simulink model "ADCS_Simulink_FSW"  (R2025b)
settings: Solver=VariableStepAuto  StartTime=8000  StopTime=8700  FixedStep=0.001  RelTol=1e-3
PreLoadFcn:
  | addpath(genpath('../'))
  | adcsModelSetup();
values from neighbouring files (symbols this model uses):
  dT_Control = 1/10    (= 0.1)    [adcsModelSetup.m]
  fNoiseOn = 0    [adcsModelSetup.m]
undefined symbols (not defined in the file or in its folder): DiscIntNeverNeededParam, IAU, juliandate
libraries: vrlib x16, simulink_extras x7, sharedtransform x5, sharedutil x4, aerolibutil x4, sFunctionLibrary x4, simulink x3, matrix_library x2, aerolibtransform2 x2
(part 1 of 2)
settings Model: Creator=prani  LastModifiedBy=palla
settings DebuggingCC: ConsistencyChecking=warning  ArrayBoundsChecking=warning  CheckMatrixSingularityMsg=warning  ParameterUnderflowMsg=error  SFcnCompatibilityMsg=warning

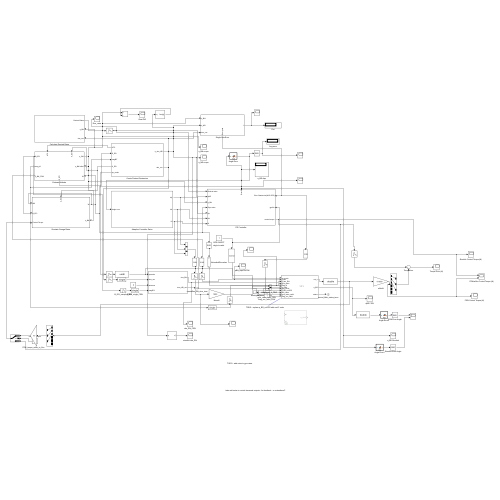
[thumbnail: Simulink's stored preview of the top-level diagram]
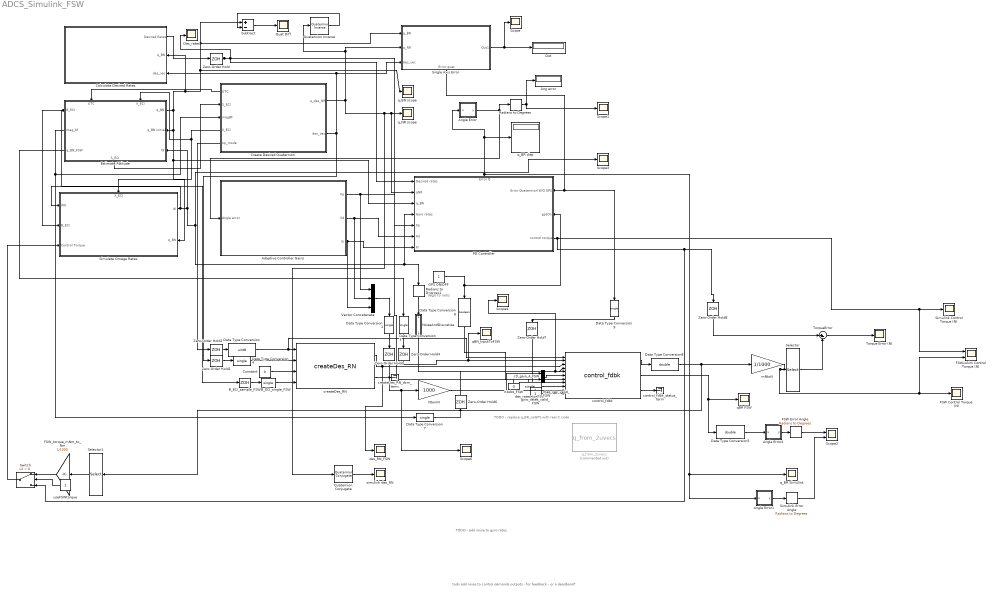
== system ADCS_Simulink_FSW ==
  note: todo add noise to control demands outputs - for feedback - or a deadband?
  note: TODO - add noise to gyro rates
  note: TODO - replace q_BR_noGPS with real C code
  note: deg/s to rad/s
  Adaptive Controller Gains : Subsystem
  Ang error : Display
  Angle Error : MATLAB Function  TreatAsAtomicUnit=on
  Angle Error1 : MATLAB Function  TreatAsAtomicUnit=on
  Angle Error2 : MATLAB Function  TreatAsAtomicUnit=on
  B_ECI_sample_FSW : ZeroOrderHold  SampleTime=dT_Control
  B_ECI_single_FSW : DataTypeConversion  OutDataTypeStr=single  SaturateOnIntegerOverflow=off  RndMeth=Floor
  Calculate Desired Rates : Subsystem
      settings: PortSchema="{\"entries\":[{\"content\":{\"sides\":[{\"content\":{},\"type\":\"ConnectorPlacement.EquallySpacedRectSide\",\"uuid\":\"787b8ffa-2bb6-4814-9cee-30d0a9949d62\"},{\"content\":{\"connectorIds\":[\"Out1\",\"In1\",\"In2\"],\"side\":\"RIGHT\"},\"type\":\"ConnectorPlacement.EquallySpacedRectSide\",\"uuid\":\"3e27d9b8-c1eb-4c63-90b1-636b0c297a4b\"},{\"content\":{\"side\":\"TOP\"},\"type\":\"ConnectorPlacement.EquallySpacedRectSide\",\"uuid\":\"66d7efb2-8eb7-483d-b673-bec0e962b7d7\"}]},\"type\":\"ConnectorPlacement.EquallySpacedConnector\",\"uuid\":\"bfb47682-ffbd-402c-af6d-784f4b216212\"}],\"packageUris\":[\"http://schema.mathworks.com/mf0/Connector/R2020b\"],\"version\":\"1.0\"}"
  Constant : Constant  Value=0  OutDataTypeStr=uint8
  Create Desired Quaternion : Subsystem
      settings: PortSchema="{\"entries\":[{\"content\":{\"sides\":[{\"content\":{\"connectorIds\":[\"Out3\",\"In1\",\"In2\",\"Out4\",\"Out5\"]},\"type\":\"ConnectorPlacement.EquallySpacedRectSide\",\"uuid\":\"a06b4b20-baa8-4cd2-8731-8e2324dbb8fc\"},{\"content\":{\"connectorIds\":[\"Out1\",\"Out2\"],\"side\":\"RIGHT\"},\"type\":\"ConnectorPlacement.EquallySpacedRectSide\",\"uuid\":\"e89e67ff-4894-42c1-b3ac-017f3fc977aa\"},{\"content\":{\"side\":\"TOP\"},\"type\":\"ConnectorPlacement.EquallySpacedRectSide\",\"uuid\":\"6ee5ea32-5253-456a-b6dd-ef60fd48a9e3\"}]},\"type\":\"ConnectorPlacement.EquallySpacedConnector\",\"uuid\":\"b732bf39-7b48-418d-8437-db30d99856db\"}],\"packageUris\":[\"http://schema.mathworks.com/mf0/Connector/R2020b\"],\"version\":\"1.0\"}"
  Data Type Conversion : DataTypeConversion  OutDataTypeStr=uint8  SaturateOnIntegerOverflow=off  RndMeth=Floor
  Data Type Conversion{1,3..4,7,9} (5 alike) : DataTypeConversion  OutDataTypeStr=single  SaturateOnIntegerOverflow=off  RndMeth=Floor
  Data Type Conversion5 : DataTypeConversion  OutDataTypeStr=double  SaturateOnIntegerOverflow=off  RndMeth=Floor
  Data Type Conversion6 : DataTypeConversion  OutDataTypeStr=boolean  SaturateOnIntegerOverflow=off  RndMeth=Floor
  Data Type Conversion8 : DataTypeConversion  OutDataTypeStr=double  SaturateOnIntegerOverflow=off  RndMeth=Floor
  Des_rates : Scope
      settings: ActiveDisplayYMinimum=-7.5812097384350083E-16  ActiveDisplayYMaximum=1.8036722603787631E-16  DataLoggingVariableName=ScopeData11
  Dot : Display
  Estimate Attitude : Subsystem
      settings: PortSchema="{\"entries\":[{\"content\":{\"sides\":[{\"content\":{\"connectorIds\":[\"Out3\",\"Out4\",\"Out5\"]},\"type\":\"ConnectorPlacement.EquallySpacedRectSide\",\"uuid\":\"9e22cb63-f739-4def-bc16-8f5ac96da1b2\"},{\"content\":{\"connectorIds\":[\"Out1\",\"In3\",\"In4\"],\"side\":\"RIGHT\"},\"type\":\"ConnectorPlacement.EquallySpacedRectSide\",\"uuid\":\"185e8ae2-f047-4dfe-b4b8-b24ace8a5036\"},{\"content\":{\"connectorIds\":[\"In1\",\"In2\"],\"side\":\"TOP\"},\"type\":\"ConnectorPlacement.EquallySpacedRectSide\",\"uuid\":\"aba5f04b-f2ef-4373-8d95-838bf2fc0f7e\"},{\"content\":{\"connectorIds\":[\"Out2\"],\"side\":\"BOTTOM\"},\"type\":\"ConnectorPlacement.EquallySpacedRectSide\",\"uuid\":\"34d3ae2b-3f47-4699-99b9-a603dee72b74\"}]},\"type\":\"ConnectorPlacement.EquallySpacedConnector\",\"uuid\":\"020a8ac0-54fe-466e-8166-8e2d9bca8ffa\"}],\"packageUris\":[\"http://schema.mathworks.com/mf0/Connector/R2020b\"],\"version\":\"1.0\"}"
  FSW Control Torque (N) : Scope
      settings: ActiveDisplayYMinimum=-0.1409447193145752  ActiveDisplayYMaximum=0.096963930130004886  DataLoggingVariableName=ScopeData30
  FSW Error Angle : simulink_extras/Transformations/Radians to Degrees
  FSW_torque_mNm_to_Nm : Gain  Gain=1/1000  OutDataTypeStr=double
  FSWvsSim Control Torque (N) : Scope  NumInputPorts=2
      settings: ActiveDisplayYMinimum=-0.021514837503433224  ActiveDisplayYMaximum=0.085270786523818975  DataLoggingVariableName=ScopeData45
  GPS ON/OFF : Constant
  Kbdot_FSW : Constant  Value=0  OutDataTypeStr=single  SampleTime=dT_Control
  NoiseAndDiscretise : Subsystem  mask{Mean=[0;0;0];, Variance=0.1*ones(3,1);, dT=dT_Control, fNoiseOn=1}
      mask prompts: fNoiseOn "Noise On (1/0)"
  NtomN : Gain  Gain=1000  OutDataTypeStr=single
  PD Controller : Subsystem
      settings: PortSchema="{\"entries\":[{\"content\":{\"sides\":[{\"content\":{\"connectorIds\":[\"In1\",\"In2\",\"In3\",\"In4\",\"In5\",\"In6\",\"In7\"]},\"type\":\"ConnectorPlacement.EquallySpacedRectSide\",\"uuid\":\"e7cfb03b-fdce-49bd-b114-b6383fec3453\"},{\"content\":{\"connectorIds\":[\"In8\",\"In9\",\"Out1\"],\"side\":\"RIGHT\"},\"type\":\"ConnectorPlacement.EquallySpacedRectSide\",\"uuid\":\"354243bd-d6fe-41fe-9aaf-62ec8dd6b288\"},{\"content\":{\"connectorIds\":[\"Out2\"],\"side\":\"TOP\"},\"type\":\"ConnectorPlacement.EquallySpacedRectSide\",\"uuid\":\"5bccfe41-e6a5-4734-99aa-97d0c6c76924\"}]},\"type\":\"ConnectorPlacement.EquallySpacedConnector\",\"uuid\":\"9d160725-4233-4f19-a31f-b456d9eba014\"}],\"packageUris\":[\"http://schema.mathworks.com/mf0/Connector/R2020b\"],\"version\":\"1.0\"}"
  Quat Diff : Scope
      settings: ActiveDisplayYMinimum=-2.4278695362681826  ActiveDisplayYMaximum=3.4846862195685198
  Quaternion Conjugate : aerolibutil/Quaternion Conjugate
  Quaternion Inverse : aerolibutil/Quaternion Inverse
  Radians to Degrees : simulink_extras/Transformations/Radians to Degrees
  Radians to Degrees1 : simulink_extras/Transformations/Radians to Degrees
  Scope{,1,3..4,6} (5 alike) : Scope
      Scope settings: ActiveDisplayYMinimum=-1.3627045234786557  ActiveDisplayYMaximum=1.3194577353207935  DataLoggingVariableName=ScopeData20
      Scope1 settings: ActiveDisplayYMinimum=-45.683444261397909  ActiveDisplayYMaximum=242.34455590666121
      Scope3 settings: ActiveDisplayYMinimum=-0.32288965159303823  ActiveDisplayYMaximum=0.19416046551698385  DataLoggingVariableName=ScopeData14
      Scope4 settings: ActiveDisplayYMinimum=-18.264092922210693  ActiveDisplayYMaximum=12.284894466400146  DataLoggingVariableName=ScopeData46
      Scope6 settings: ActiveDisplayYMinimum=-0.062499999999999986  ActiveDisplayYMaximum=0.5625  DataLoggingVariableName=ScopeData32
  Scope2 : Scope  NumInputPorts=2
      settings: ActiveDisplayYMinimum=-18.982567049476042  ActiveDisplayYMaximum=182.17965657034267  DataLoggingVariableName=ScopeData36
  Selector : Selector  InputPortWidth=6  IndexOptions=Index vector (dialog)  Indices=[1 2 3]  OutputSizes=1
  Selector1 : Selector  InputPortWidth=6  IndexOptions=Index vector (dialog)  Indices=[1 2 3]  OutputSizes=1
  Simulate Omega Rates : Subsystem
      settings: PortSchema="{\"entries\":[{\"content\":{\"sides\":[{\"content\":{\"connectorIds\":[\"In1\",\"In2\",\"In3\"]},\"type\":\"ConnectorPlacement.EquallySpacedRectSide\",\"uuid\":\"e90ec8a0-4b74-4e10-b2a7-e5fd2ae1e771\"},{\"content\":{\"connectorIds\":[\"Out1\",\"In5\"],\"side\":\"RIGHT\"},\"type\":\"ConnectorPlacement.EquallySpacedRectSide\",\"uuid\":\"99d2540c-d7ae-4cc6-9c8c-9f3376bc2204\"},{\"content\":{\"connectorIds\":[\"In4\"],\"side\":\"TOP\"},\"type\":\"ConnectorPlacement.EquallySpacedRectSide\",\"uuid\":\"1bb08a9c-3229-4768-9d5b-a9b542d9af4a\"},{\"content\":{\"side\":\"BOTTOM\"},\"type\":\"ConnectorPlacement.EquallySpacedRectSide\",\"uuid\":\"162a9998-95a8-4725-8cf6-c5c7f5c27aaf\"}]},\"type\":\"ConnectorPlacement.EquallySpacedConnector\",\"uuid\":\"560ef827-5a28-40b0-8e31-165022fcc335\"}],\"packageUris\":[\"http://schema.mathworks.com/mf0/Connector/R2020b\"],\"version\":\"1.0\"}"
  Simulink Control Torque (N) : Scope
      settings: ActiveDisplayYMinimum=-0.19285196494450457  ActiveDisplayYMaximum=0.22481895277845004  DataLoggingVariableName=ScopeData6
  Simulink Error Angle : simulink_extras/Transformations/Radians to Degrees
  Single Axis Error : Subsystem
      settings: PortSchema="{\"entries\":[{\"content\":{\"sides\":[{\"content\":{\"connectorIds\":[\"In1\",\"In2\",\"In3\"]},\"type\":\"ConnectorPlacement.EquallySpacedRectSide\",\"uuid\":\"b8267f91-c5e3-4d33-8203-7c1a132bc190\"},{\"content\":{\"connectorIds\":[\"Out1\"],\"side\":\"RIGHT\"},\"type\":\"ConnectorPlacement.EquallySpacedRectSide\",\"uuid\":\"66851e38-bd34-4725-8451-fc4e99cb0cf9\"},{\"content\":{\"side\":\"TOP\"},\"type\":\"ConnectorPlacement.EquallySpacedRectSide\",\"uuid\":\"dfe73cc2-180d-42b0-a8bc-469053aa0085\"},{\"content\":{\"connectorIds\":[\"Out2\"],\"side\":\"BOTTOM\"},\"type\":\"ConnectorPlacement.EquallySpacedRectSide\",\"uuid\":\"e4419c1d-78c1-4c02-89c9-5404581220d5\"}]},\"type\":\"ConnectorPlacement.EquallySpacedConnector\",\"uuid\":\"596ae20b-822c-4bb8-8293-fd61ff3bd564\"}],\"packageUris\":[\"http://schema.mathworks.com/mf0/Connector/R2020b\"],\"version\":\"1.0\"}"
  Subtract : Sum  Inputs=+-
  Switch : Switch  Criteria=u2 > Threshold  SaturateOnIntegerOverflow=off  InputSameDT=off
  Torque Error (N) : Scope
      settings: ActiveDisplayYMinimum=-0.015390724559551172  ActiveDisplayYMaximum=0.017866098622383832  DataLoggingVariableName=ScopeData31
  TorqueError : Sum  Inputs=|+-
  Vector Concatenate : Concatenate  NumInputs=3
  Zero-Order Hold : ZeroOrderHold
  Zero-Order Hold{1..4,6..8} (7 alike) : ZeroOrderHold  SampleTime=dT_Control
  control_fdbk : sFunctionLibrary/control_fdbk  SystemSampleTime=-1  VariantActivationTime=update diagram  EmptyChoice=off  PassThrough=off  PassThroughVariantControl=(default)  EmptyChoiceVariantControl=(default)  AllowFlexibleInterface=on  Latency=0  AutoFrameSizeCalculation=off
  control_fdbk_status_term : Terminator
  createDes_RN : sFunctionLibrary/createDes_RN  SystemSampleTime=-1  VariantActivationTime=update diagram  EmptyChoice=off  PassThrough=off  PassThroughVariantControl=(default)  EmptyChoiceVariantControl=(default)  AllowFlexibleInterface=on  Latency=0  AutoFrameSizeCalculation=off
  createDes_RN_dcm_term : Terminator
  ctl_gain_4_FSW : Concatenate
  des_RN_FSW : Scope
      settings: ActiveDisplayYMinimum=-1.2834040716711121  ActiveDisplayYMaximum=1.1693099245008391  DataLoggingVariableName=ScopeData33
  des_rates_to_FSW : DataTypeConversion  OutDataTypeStr=single  SaturateOnIntegerOverflow=off  RndMeth=Floor
  gyro_rates_valid_FSW : Constant  OutDataTypeStr=int32  SampleTime=dT_Control
  mNtoN : Gain  Gain=1/1000  OutDataTypeStr=double
  mag_vec_valid_FSW : Constant  OutDataTypeStr=int32  SampleTime=dT_Control
  qBN_InputToFSW : Scope
      settings: ActiveDisplayYMinimum=-1.1772833690047264  ActiveDisplayYMaximum=1.2419203743338585  DataLoggingVariableName=ScopeData41
  qBR FSW : Scope
      settings: ActiveDisplayYMinimum=-0.87164634466171265  ActiveDisplayYMaximum=1.2077648043632507  DataLoggingVariableName=ScopeData35
  q_BN scope : Scope
      settings: ActiveDisplayYMinimum=-1.3505009914765778  ActiveDisplayYMaximum=1.1663107803216415  DataLoggingVariableName=ScopeData4
  q_BR Simulink : Scope
      settings: ActiveDisplayYMinimum=-0.87279489122515741  ActiveDisplayYMaximum=1.2079931709273608  DataLoggingVariableName=ScopeData28
  q_BR disp : Display
  q_NR scope : Scope
      settings: ActiveDisplayYMinimum=-0.18271803790267854  ActiveDisplayYMaximum=0.94151609942253189  DataLoggingVariableName=ScopeData18
  q_from_2uvecs : sFunctionLibrary/q_from_2uvecs  Commented=on  SystemSampleTime=-1  VariantActivationTime=update diagram  EmptyChoice=off  PassThrough=off  PassThroughVariantControl=(default)  EmptyChoiceVariantControl=(default)  AllowFlexibleInterface=on  Latency=0  AutoFrameSizeCalculation=off
  simulink des_RN : Scope
      settings: ActiveDisplayYMinimum=-1.2267552075477972  ActiveDisplayYMaximum=1.2259656861469523  DataLoggingVariableName=ScopeData34
  useFSWtorque : Constant
  wires:
  Simulate Omega Rates/1(W) -> Scope3/1, PD Controller/4(Gyro rates), Radians to Degrees1/1, Estimate Attitude/4(W), Simulate Omega Rates/1(W0)
  Create Desired Quaternion/1(q_des_NR) -> Single Axis Error/2(q_NR), Quaternion Inverse/1, Quaternion Conjugate/1, q_NR scope/1, PD Controller/2(qNR)
  Single Axis Error/1(Out1) -> Scope/1, Dot/1
  Calculate Desired Rates/1(Desired Rates) -> Zero-Order Hold/1
  Adaptive Controller Gains/1(Kp) -> Vector Concatenate/1, PD Controller/5(Kp)
  Adaptive Controller Gains/2(Kd) -> Vector Concatenate/2, PD Controller/6(Kd)
  Adaptive Controller Gains/3(Ki) -> Vector Concatenate/3, PD Controller/7(Ki)
  Radians to Degrees/1 -> Scope1/1, Ang error/1
  Estimate Attitude/1(q_BN) -> PD Controller/3(q_BN), Simulate Omega Rates/5(q_BN), Estimate Attitude/3(q_BN initial), Calculate Desired Rates/1(q_BN), Subtract/1, Single Axis Error/1(q_BN), q_BN scope/1
  Quaternion Inverse/1 -> Subtract/2
  Subtract/1 -> Quat Diff/1
  Zero-Order Hold/1 -> Des_rates/1, PD Controller/1(Desired rates), des_rates_to_FSW/1
  Single Axis Error/2(Error quat) -> Data Type Conversion9/1, PD Controller/8(Error Quaternion(W/O GPS))
  Create Desired Quaternion/4(X_ECI) -> Estimate Attitude/2(X_ECI), Simulate Omega Rates/4(X_ECI)
  Create Desired Quaternion/3(UTC) -> Estimate Attitude/1(UTC)
  Estimate Attitude/2(S_ECI) -> Create Desired Quaternion/1(S_ECI)
  Create Desired Quaternion/2(des_vec) -> Single Axis Error/3(des_vec), Calculate Desired Rates/2(des_vec), Zero-Order Hold1/1
  Estimate Attitude/3(B_ECI) -> Simulate Omega Rates/2("B_ECI "), B_ECI_sample_FSW/1
  Create Desired Quaternion/5(op_mode) -> Zero-Order Hold2/1
  createDes_RN/1 -> des_RN_FSW/1, control_fdbk/3
  Vector Concatenate/1 -> Data Type Conversion1/1
  Angle Error/1(y) -> Radians to Degrees/1, Adaptive Controller Gains/1(Angle error)
  control_fdbk/1 -> Data Type Conversion8/1
  Data Type Conversion/1 -> createDes_RN/1, control_fdbk/1
  Data Type Conversion1/1 -> Zero-Order Hold3/1
  Data Type Conversion3/1 -> Zero-Order Hold4/1
  Zero-Order Hold1/1 -> Data Type Conversion4/1
  Zero-Order Hold2/1 -> Data Type Conversion/1
  Zero-Order Hold3/1 -> Scope6/1, NtomN/1
  Zero-Order Hold4/1 -> qBN_InputToFSW/1, control_fdbk/2
  Zero-Order Hold8/1 -> TorqueError/1
  TorqueError/1 -> Torque Error (N)/1
  Estimate Attitude/4(mag_bf) -> Create Desired Quaternion/2(magBF), Data Type Conversion7/1
  Data Type Conversion7/1 -> Zero-Order Hold6/1
  Data Type Conversion8/1 -> Selector1/1, mNtoN/1
  Quaternion Conjugate/1 -> simulink des_RN/1
  Data Type Conversion4/1 -> createDes_RN/2
  Constant/1 -> createDes_RN/3
  Zero-Order Hold6/1 -> control_fdbk/5
  control_fdbk/2 -> qBR FSW/1, Data Type Conversion5/1
  mNtoN/1 -> FSWvsSim Control Torque (N)/2, FSW Control Torque (N)/1, Selector/1
  Selector/1 -> TorqueError/2
  Angle Error2/1(y) -> FSW Error Angle/1
  Angle Error1/1(y) -> Simulink Error Angle/1
  Simulink Error Angle/1 -> Scope2/2
  FSW Error Angle/1 -> Scope2/1
  Data Type Conversion5/1 -> Angle Error2/1(u)
  NoiseAndDiscretise/1(Out1) -> Scope4/1, control_fdbk/4
  Radians to Degrees1/1 -> NoiseAndDiscretise/1(In1)
  Estimate Attitude/5(q_BN_FSW) -> Data Type Conversion3/1
  PD Controller/1(control torque) -> FSWvsSim Control Torque (N)/1, Simulink Control Torque (N)/1, Switch/3, Zero-Order Hold8/1
  GPS ON/OFF/1 -> Data Type Conversion6/1, PD Controller/9(gpsOn)
  Data Type Conversion6/1 -> control_fdbk/7
  PD Controller/2(Error Q) -> q_BR Simulink/1, Angle Error1/1(u), Angle Error/1(u), q_BR disp/1
  Zero-Order Hold7/1 -> control_fdbk/8
  Data Type Conversion9/1 -> Zero-Order Hold7/1
  Switch/1 -> Simulate Omega Rates/3(Control Torque)
  useFSWtorque/1 -> Switch/2
  des_rates_to_FSW/1 -> control_fdbk/9
  gyro_rates_valid_FSW/1 -> control_fdbk/10
  mag_vec_valid_FSW/1 -> control_fdbk/11
  control_fdbk/3 -> control_fdbk_status_term/1
  createDes_RN/2 -> createDes_RN_dcm_term/1
  NtomN/1 -> ctl_gain_4_FSW/1
  Kbdot_FSW/1 -> ctl_gain_4_FSW/2
  ctl_gain_4_FSW/1 -> control_fdbk/6
  B_ECI_sample_FSW/1 -> B_ECI_single_FSW/1
  B_ECI_single_FSW/1 -> createDes_RN/4
  Selector1/1 -> FSW_torque_mNm_to_Nm/1
  FSW_torque_mNm_to_Nm/1 -> Switch/1

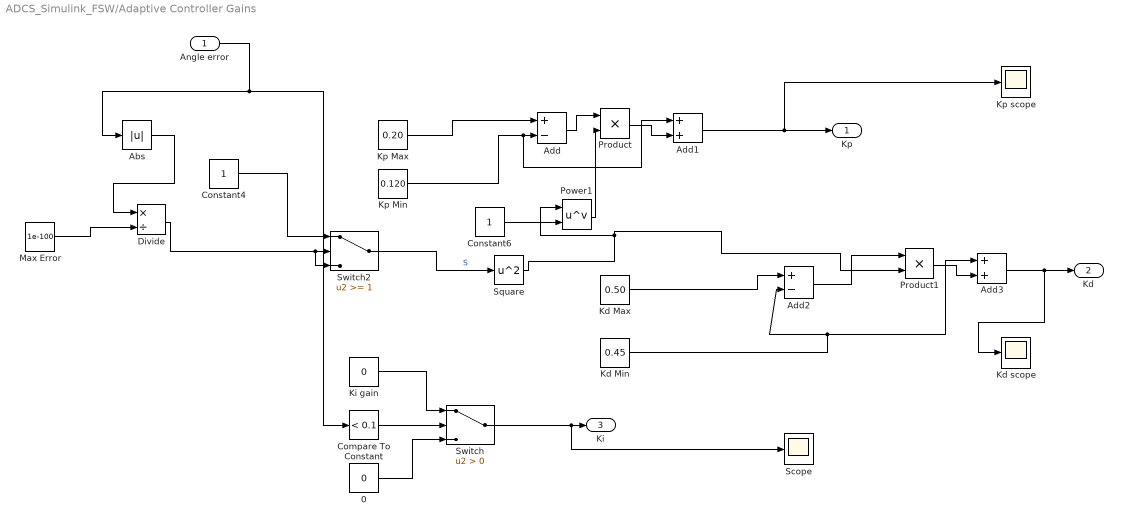
== system ADCS_Simulink_FSW/Adaptive Controller Gains ==
  Angle error : Inport
  0 : Constant  Value=0
  Abs : Abs  SaturateOnIntegerOverflow=off
  Add : Sum  Inputs=+-
  Add1 : Sum
  Add2 : Sum  Inputs=+-
  Add3 : Sum
  Compare To Constant : simulink/Logic and Bit Operations/Compare To Constant  relop=<  const=0.1  OutDataTypeStr=boolean
  Constant4 : Constant
  Constant6 : Constant
  Divide : Product  Inputs=*/
  Kd Max : Constant  Value=0.50
  Kd Min : Constant  Value=0.45
  Kd scope : Scope
      settings: ActiveDisplayYMinimum=0.4  ActiveDisplayYMaximum=0.6  DataLoggingVariableName=ScopeData3
  Ki gain : Constant  Value=0
  Kp Max : Constant  Value=0.20  VectorParams1D=off
  Kp Min : Constant  Value=0.120
  Kp scope : Scope
      settings: ActiveDisplayYMinimum=0.1  ActiveDisplayYMaximum=0.30000000000000004  DataLoggingVariableName=ScopeData5
  Max Error : Constant  Value=1e-100
  Power1 : Math  Operator=pow
  Product : Product
  Product1 : Product
  Scope : Scope
      settings: DataLoggingVariableName=ScopeData2
  Square : Math  Operator=square
  Switch : Switch  Criteria=u2 > Threshold  SaturateOnIntegerOverflow=off  InputSameDT=off
  Switch2 : Switch  Threshold=1  SaturateOnIntegerOverflow=off  InputSameDT=off
  Kp : Outport
  Kd : Outport  Port=2
  Ki : Outport  Port=3
  wires:
  Angle error/1 -> Compare To Constant/1, Abs/1
  Max Error/1 -> Divide/2
  Constant4/1 -> Switch2/1
  Kp Max/1 -> Add/1
  Kp Min/1 -> Add1/1, Add/2
  Add/1 -> Product/1
  Product/1 -> Add1/2
  Kd Min/1 -> Add3/1, Add2/2
  Product1/1 -> Add3/2
  Kd Max/1 -> Add2/1
  Add2/1 -> Product1/1
  Abs/1 -> Divide/1
  Add3/1 -> Kd/1, Kd scope/1
  Add1/1 -> Kp scope/1, Kp/1
  Constant6/1 -> Power1/2
  Power1/1 -> Product/2
  Switch2/1 -> Square/1  "S"
  Compare To Constant/1 -> Switch/2
  Ki gain/1 -> Switch/1
  0/1 -> Switch/3
  Switch/1 -> Scope/1, Ki/1
  Divide/1 -> Switch2/3, Switch2/2
  Square/1 -> Product1/2, Power1/1

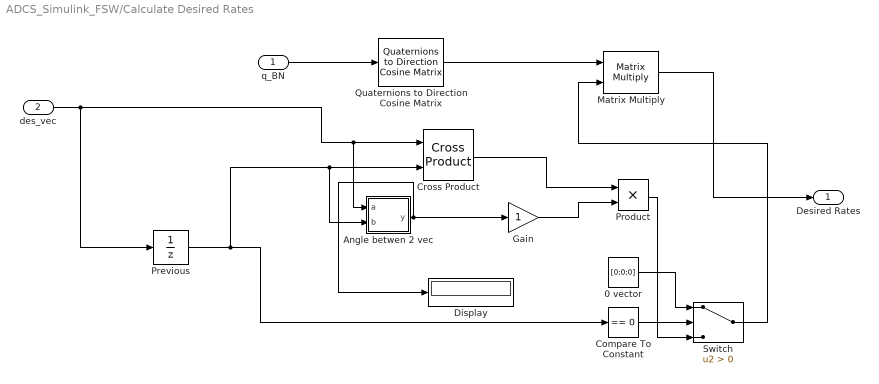
== system ADCS_Simulink_FSW/Calculate Desired Rates ==
  q_BN : Inport
  des_vec : Inport  Port=2
  0 vector : Constant  Value=[0;0;0]
  Angle betwen 2 vec : MATLAB Function  TreatAsAtomicUnit=on
  Compare To Constant : simulink/Logic and Bit Operations/Compare To Constant  relop===  const=0  OutDataTypeStr=boolean
  Cross Product : matrix_library/Cross Product
  Display : Display
  Gain : Gain
  Matrix Multiply : Product  Multiplication=Matrix(*)
  Previous : UnitDelay  InitialCondition=[0; 0; 0]  SampleTime=-1  HasFrameUpgradeWarning=on
  Product : Product
  Quaternions to Direction Cosine Matrix : sharedtransform/Quaternions to  Direction Cosine Matrix  aMode=aMode
      settings: LibrarySourceBlock=|
      | aerolibtransform2/Quaternions to
      | Direction Cosine Matrix
  Switch : Switch  Criteria=u2 > Threshold  SaturateOnIntegerOverflow=off  InputSameDT=off
  Desired Rates : Outport
  wires:
  Angle betwen 2 vec/1(y) -> Display/1, Gain/1
  Previous/1 -> Compare To Constant/1, Cross Product/2, Angle betwen 2 vec/2(b)
  Gain/1 -> Product/2
  Cross Product/1 -> Product/1
  Product/1 -> Switch/3
  des_vec/1 -> Previous/1, Angle betwen 2 vec/1(a), Cross Product/1
  0 vector/1 -> Switch/1
  Compare To Constant/1 -> Switch/2
  Switch/1 -> Matrix Multiply/2
  q_BN/1 -> Quaternions to Direction Cosine Matrix/1
  Quaternions to Direction Cosine Matrix/1 -> Matrix Multiply/1
  Matrix Multiply/1 -> Desired Rates/1

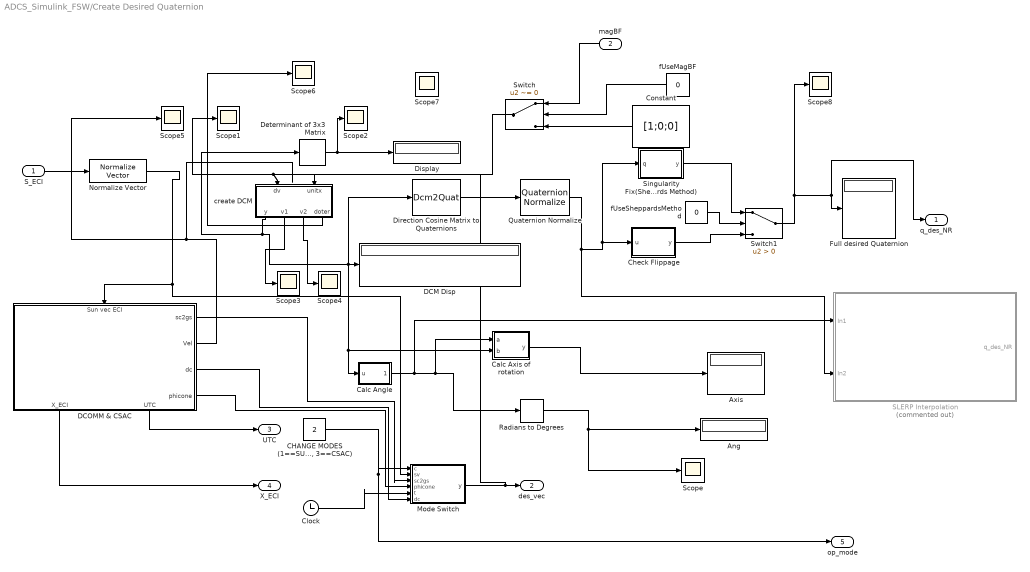
== system ADCS_Simulink_FSW/Create Desired Quaternion ==
  S_ECI : Inport
  magBF : Inport  Port=2
  Ang : Display
  Axis : Display
  "CHANGE MODES (1==SUN, 2==DCOMM, 3==CSAC)" : Constant  Value=2
  Calc Angle : MATLAB Function  TreatAsAtomicUnit=on
  Calc Axis of rotation : MATLAB Function  TreatAsAtomicUnit=on
  Check Flippage : MATLAB Function  TreatAsAtomicUnit=on
  Clock : Clock
  Constant : Constant  Value=[1;0;0]  VectorParams1D=off
  DCM Disp : Display
  DCOMM & CSAC : Subsystem
      settings: PortSchema="{\"entries\":[{\"content\":{\"sides\":[{\"content\":{},\"type\":\"ConnectorPlacement.EquallySpacedRectSide\",\"uuid\":\"787b8ffa-2bb6-4814-9cee-30d0a9949d62\"},{\"content\":{\"connectorIds\":[\"Out1\",\"Out2\",\"Out3\",\"Out4\"],\"side\":\"RIGHT\"},\"type\":\"ConnectorPlacement.EquallySpacedRectSide\",\"uuid\":\"3e27d9b8-c1eb-4c63-90b1-636b0c297a4b\"},{\"content\":{\"connectorIds\":[\"In1\"],\"side\":\"TOP\"},\"type\":\"ConnectorPlacement.EquallySpacedRectSide\",\"uuid\":\"66d7efb2-8eb7-483d-b673-bec0e962b7d7\"},{\"content\":{\"connectorIds\":[\"Out5\",\"Out6\"],\"side\":\"BOTTOM\"},\"type\":\"ConnectorPlacement.EquallySpacedRectSide\",\"uuid\":\"f2142c7a-e9b1-4676-9442-99b79bc541a0\"}]},\"type\":\"ConnectorPlacement.EquallySpacedConnector\",\"uuid\":\"bfb47682-ffbd-402c-af6d-784f4b216212\"}],\"packageUris\":[\"http://schema.mathworks.com/mf0/Connector/R2020b\"],\"version\":\"1.0\"}"
  Determinant of 3x3 Matrix : sharedutil/Determinant of 3x3 Matrix  aMode=aMode
      settings: LibrarySourceBlock=|
      | aerolibutil/Determinant of
      | 3x3 Matrix
  Direction Cosine Matrix to Quaternions : Dcm2Quat
  Display : Display
  Full desired Quaternion : Display
  Mode Switch : MATLAB Function  TreatAsAtomicUnit=on
  Normalize Vector : vrlib/Utilities/Normalize Vector  maxzero=0
  Quaternion Normalize : sharedutil/Quaternion Normalize  aMode=aMode
  Radians to Degrees : simulink_extras/Transformations/Radians to Degrees
  SLERP Interpolation : Subsystem  Commented=on
  Scope{,1..8} (9 alike) : Scope
      Scope settings: ActiveDisplayYMinimum=54.843753253763992  ActiveDisplayYMaximum=243.09394752220919  DataLoggingVariableName=ScopeData19
      Scope1 settings: ActiveDisplayYMinimum=-2.4642997600105518  ActiveDisplayYMaximum=0.88408956918614268  DataLoggingVariableName=ScopeData8
      Scope2 settings: ActiveDisplayYMinimum=0.99999999995780953  ActiveDisplayYMaximum=1.0000000000475318  DataLoggingVariableName=ScopeData3
      Scope3 settings: ActiveDisplayYMinimum=-3.0436341558557145  ActiveDisplayYMaximum=1.5557132316836486  DataLoggingVariableName=ScopeData21
      Scope4 settings: ActiveDisplayYMinimum=-0.39677371902603914  ActiveDisplayYMaximum=1.0300816259123484  DataLoggingVariableName=ScopeData22
      Scope5 settings: ActiveDisplayYMinimum=-3863.6885466348626  ActiveDisplayYMaximum=7764.3844723641732  DataLoggingVariableName=ScopeData23
      Scope6 settings: ActiveDisplayYMinimum=-0.597873861939996  ActiveDisplayYMaximum=1.0836231729395602  DataLoggingVariableName=ScopeData24
      Scope7 settings: ActiveDisplayYMinimum=-1  ActiveDisplayYMaximum=1  DataLoggingVariableName=ScopeData25
      Scope8 settings: ActiveDisplayYMinimum=-0.86317029227862363  ActiveDisplayYMaximum=1.057535107720678  DataLoggingVariableName=ScopeData50
  Singularity Fix(Sheppards Method) : MATLAB Function  TreatAsAtomicUnit=on
  Switch : Switch  Criteria=u2 ~= 0  SaturateOnIntegerOverflow=off  InputSameDT=off
  Switch1 : Switch  Criteria=u2 > Threshold  SaturateOnIntegerOverflow=off  InputSameDT=off
  create DCM : MATLAB Function  TreatAsAtomicUnit=on
  fUseMagBF : Constant  Value=0
  fUseSheppardsMethod : Constant  Value=0
  q_des_NR : Outport
  des_vec : Outport  Port=2
  UTC : Outport  Port=3
  X_ECI : Outport  Port=4
  op_mode : Outport  Port=5
  wires:
  Determinant of 3x3 Matrix/1 -> Scope2/1, Display/1
  Quaternion Normalize/1 -> Singularity Fix(Sheppards Method)/1(q), Check Flippage/1(u), SLERP Interpolation/2(In2)
  DCOMM & CSAC/1(sc2gs) -> Mode Switch/3(sc2gs)
  DCOMM & CSAC/4(phicone) -> Mode Switch/4(phicone)
  Normalize Vector/1 -> Mode Switch/2(sv), DCOMM & CSAC/1(Sun vec ECI)
  Calc Angle/1(angle) -> SLERP Interpolation/1(In1), Radians to Degrees/1, Calc Axis of rotation/1(a)
  Calc Axis of rotation/1(y) -> Axis/1
  Radians to Degrees/1 -> Scope/1, Ang/1
  Switch1/1 -> q_des_NR/1, Full desired Quaternion/1, Scope8/1
  "CHANGE MODES (1==SUN, 2==DCOMM, 3==CSAC)"/1 -> op_mode/1, Mode Switch/1(c)
  Mode Switch/1(y) -> Scope1/1, create DCM/1(dv), des_vec/1
  DCOMM & CSAC/6(UTC) -> UTC/1
  DCOMM & CSAC/5(X_ECI) -> X_ECI/1
  Clock/1 -> Mode Switch/5(t)
  Direction Cosine Matrix to Quaternions/1 -> Quaternion Normalize/1
  S_ECI/1 -> Normalize Vector/1
  DCOMM & CSAC/3(dc) -> Mode Switch/6(dc)
  create DCM/1(y) -> Direction Cosine Matrix to Quaternions/1, DCM Disp/1, Calc Angle/1(u), Calc Axis of rotation/2(b), Determinant of 3x3 Matrix/1
  create DCM/2(v1) -> Scope3/1
  create DCM/3(v2) -> Scope4/1
  DCOMM & CSAC/2(Vel) -> Scope5/1
  create DCM/4(doter) -> Scope6/1
  ? -> Scope7/1
  Constant/1 -> Switch/3
  magBF/1 -> Switch/1
  Switch/1 -> create DCM/2(unitx)
  fUseMagBF/1 -> Switch/2
  Singularity Fix(Sheppards Method)/1(y) -> Switch1/1
  fUseSheppardsMethod/1 -> Switch1/2
  Check Flippage/1(y) -> Switch1/3

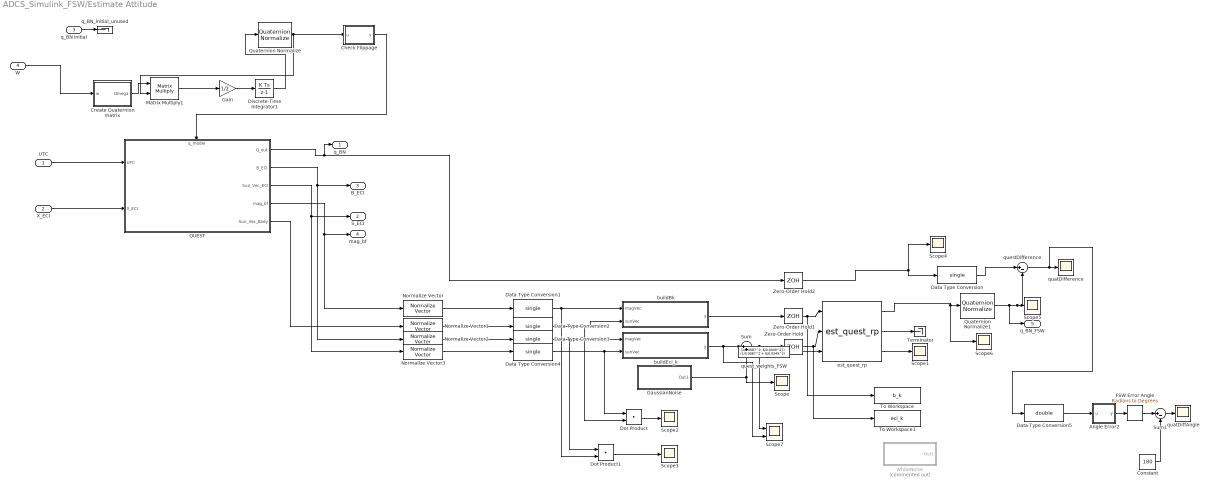
== system ADCS_Simulink_FSW/Estimate Attitude ==
  UTC : Inport
  X_ECI : Inport  Port=2
  q_BN initial : Inport  Port=3
  W : Inport  Port=4
  Angle Error2 : MATLAB Function  TreatAsAtomicUnit=on
  Check Flippage : MATLAB Function  TreatAsAtomicUnit=on
  Constant : Constant  Value=180
  Create Quaternion matrix : MATLAB Function  TreatAsAtomicUnit=on
  Data Type Conversion{,1..4} (5 alike) : DataTypeConversion  OutDataTypeStr=single  SaturateOnIntegerOverflow=off  RndMeth=Floor
  Data Type Conversion5 : DataTypeConversion  OutDataTypeStr=double  SaturateOnIntegerOverflow=off  RndMeth=Floor
  Discrete-Time Integrator1 : DiscreteIntegrator  gainval=1  InitialCondition=[1; 0 ;0; 0]  SampleTime=0.1  ICPrevOutput=DiscIntNeverNeededParam  ICPrevScaledInput=DiscIntNeverNeededParam
  Dot Product : DotProduct  OutDataTypeStr=Inherit: Inherit via internal rule
  Dot Product1 : DotProduct  OutDataTypeStr=Inherit: Inherit via internal rule
  FSW Error Angle : simulink_extras/Transformations/Radians to Degrees
  Gain : Gain  Gain=1/2
  GaussianNoise : Subsystem  mask{Mean=[0 0; 0 0; 0 0];, Variance=[1E-5 1E-5; 1E-5 1E-5; 1E-5 1E-5];, dT=dT_Control, fUseNoise=fNoiseOn}
      mask prompts: dT "Sample Rate"
  Matrix Multiply1 : Product  Multiplication=Matrix(*)
  Normalize Vector{,1..3} (4 alike) : vrlib/Utilities/Normalize Vector  maxzero=0
  QUEST : Subsystem
      settings: PortSchema="{\"entries\":[{\"content\":{\"sides\":[{\"content\":{\"connectorIds\":[\"In1\",\"In2\"]},\"type\":\"ConnectorPlacement.EquallySpacedRectSide\",\"uuid\":\"d9c028fa-a02f-4cb7-9f20-ffb15f38696f\"},{\"content\":{\"connectorIds\":[\"Out1\",\"Out2\",\"Out3\",\"Out4\",\"Out5\"],\"side\":\"RIGHT\"},\"type\":\"ConnectorPlacement.EquallySpacedRectSide\",\"uuid\":\"b35fd987-9710-478a-a6a2-9a386e56d3f0\"},{\"content\":{\"connectorIds\":[\"In3\"],\"side\":\"TOP\"},\"type\":\"ConnectorPlacement.EquallySpacedRectSide\",\"uuid\":\"048a4d82-b6fc-492d-bc3d-399353d1cfa9\"}]},\"type\":\"ConnectorPlacement.EquallySpacedConnector\",\"uuid\":\"63c844ef-071a-4ae7-9bff-0e02f454db7e\"}],\"packageUris\":[\"http://schema.mathworks.com/mf0/Connector/R2020b\"],\"version\":\"1.0\"}"
  Quaternion Normalize : sharedutil/Quaternion Normalize  aMode=aMode
  Quaternion Normalize1 : sharedutil/Quaternion Normalize  aMode=aMode
  Scope{,1..6} (7 alike) : Scope
      Scope settings: ActiveDisplayYMinimum=-0.095734192058444023  ActiveDisplayYMaximum=0.091843096539378166  DataLoggingVariableName=ScopeData48
      Scope1 settings: ActiveDisplayYMinimum=0.9  ActiveDisplayYMaximum=1.1  DataLoggingVariableName=ScopeData38
      Scope2 settings: ActiveDisplayYMinimum=0.0092174992896616459  ActiveDisplayYMaximum=0.019159605260938406  DataLoggingVariableName=ScopeData39
      Scope3 settings: ActiveDisplayYMinimum=0.55723564326763153  ActiveDisplayYMaximum=0.56547494232654572  DataLoggingVariableName=ScopeData40
      Scope4 settings: ActiveDisplayYMinimum=-0.946074689028379  ActiveDisplayYMaximum=1.2162305210031532  DataLoggingVariableName=ScopeData42
      Scope5 settings: ActiveDisplayYMinimum=-0.91803713142871857  ActiveDisplayYMaximum=1.2131121903657913  DataLoggingVariableName=ScopeData37
      Scope6 settings: ActiveDisplayYMinimum=-0.73043476045131683  ActiveDisplayYMaximum=1.772125706076622  DataLoggingVariableName=ScopeData47
  Scope7 : Scope  NumInputPorts=2
      settings: ActiveDisplayYMinimum=-9.927884615384615  ActiveDisplayYMaximum=10.072115384615385  DataLoggingVariableName=ScopeData49
  Sum : Sum  Inputs=|++
  Sum1 : Sum  Inputs=|+-
  Terminator : Terminator
  To Workspace : ToWorkspace  VariableName=b_k  SaveFormat=Timeseries  SampleTime=-1
  To Workspace1 : ToWorkspace  VariableName=eci_k  SaveFormat=Timeseries  SampleTime=-1
  WhiteNoise : Subsystem  Commented=on  mask{NoisePower=[0.1; 0.1; 0.1];, dT=0.1}
      mask prompts: NoisePower "Noise Power"; dT "Sample Rate"
  Zero-Order Hold : ZeroOrderHold  SampleTime=dT_Control
  Zero-Order Hold1 : ZeroOrderHold  SampleTime=dT_Control
  Zero-Order Hold2 : ZeroOrderHold  SampleTime=dT_Control
  buildBk : MATLAB Function  TreatAsAtomicUnit=on
  buildEci_k : MATLAB Function  TreatAsAtomicUnit=on
  est_quest_rp : sFunctionLibrary/est_quest_rp  SystemSampleTime=-1  VariantActivationTime=update diagram  EmptyChoice=off  PassThrough=off  PassThroughVariantControl=(default)  EmptyChoiceVariantControl=(default)  AllowFlexibleInterface=on  Latency=0  AutoFrameSizeCalculation=off
  q_BN_initial_unused : Terminator
  quatDiffAngle : Scope
      settings: ActiveDisplayYMinimum=-3.7566040422376545E-5  ActiveDisplayYMaximum=3.0735851257901459E-5  DataLoggingVariableName=ScopeData44
  quatDifference : Scope
      settings: ActiveDisplayYMinimum=-0.0038123510312289  ActiveDisplayYMaximum=0.0064584303181618452  DataLoggingVariableName=ScopeData43
  questDifference : Sum  Inputs=|+-
  quest_weights_FSW : Constant  Value=[1/0.0087^2; 6/0.0349^2] / (1/0.0087^2 + 6/0.0349^2)  VectorParams1D=off  OutDataTypeStr=single  SampleTime=dT_Control
  q_BN : Outport
  S_ECI : Outport  Port=2
  B_ECI : Outport  Port=3
  mag_bf : Outport  Port=4
  q_BN_FSW : Outport  Port=5
  wires:
  Discrete-Time Integrator1/1 -> Quaternion Normalize/1
  Matrix Multiply1/1 -> Gain/1
  Gain/1 -> Discrete-Time Integrator1/1
  Create Quaternion matrix/1(Omega) -> Matrix Multiply1/1
  W/1 -> Create Quaternion matrix/1(w)
  Quaternion Normalize/1 -> Check Flippage/1(u), Matrix Multiply1/2
  Check Flippage/1(y) -> QUEST/3(q_model)
  UTC/1 -> QUEST/1(UTC)
  X_ECI/1 -> QUEST/2(X_ECI)
  QUEST/1(Q_out) -> Zero-Order Hold2/1, q_BN/1
  est_quest_rp/2 -> Terminator/1
  est_quest_rp/3 -> Scope1/1
  buildEci_k/1(y) -> Scope7/2, Sum/1
  buildBk/1(y) -> Zero-Order Hold1/1
  Zero-Order Hold1/1 -> To Workspace/1, est_quest_rp/1
  QUEST/4(mag_bf) -> Normalize Vector/1, mag_bf/1
  QUEST/5(Sun_Vec_Body) -> Normalize Vector1/1
  QUEST/3(Sun_Vec_ECI) -> Normalize Vector3/1, S_ECI/1
  Dot Product/1 -> Scope2/1
  Dot Product1/1 -> Scope3/1
  QUEST/2(B_ECI) -> Normalize Vector2/1, B_ECI/1
  Data Type Conversion1/1 -> Dot Product1/2, buildBk/1(magVec)
  Data Type Conversion2/1 -> Dot Product/2, buildBk/2(sunVec)
  Data Type Conversion4/1 -> Dot Product/1, buildEci_k/2(sunVec)
  Data Type Conversion3/1 -> Dot Product1/1, buildEci_k/1(magVec)
  Normalize Vector/1 -> Data Type Conversion1/1
  Normalize Vector1/1 -> Data Type Conversion2/1
  Normalize Vector2/1 -> Data Type Conversion3/1
  Normalize Vector3/1 -> Data Type Conversion4/1
  Zero-Order Hold2/1 -> Data Type Conversion/1, Scope4/1
  Quaternion Normalize1/1 -> q_BN_FSW/1, questDifference/2, Scope5/1
  est_quest_rp/1 -> Scope6/1, Quaternion Normalize1/1
  Zero-Order Hold/1 -> To Workspace1/1, est_quest_rp/2
  Data Type Conversion5/1 -> Angle Error2/1(u)
  questDifference/1 -> Data Type Conversion5/1, quatDifference/1
  FSW Error Angle/1 -> Sum1/1
  Angle Error2/1(y) -> FSW Error Angle/1
  Sum1/1 -> quatDiffAngle/1
  Constant/1 -> Sum1/2
  Data Type Conversion/1 -> questDifference/1
  GaussianNoise/1(Out1) -> Scope/1, Sum/2
  Sum/1 -> Scope7/1, Zero-Order Hold/1
  quest_weights_FSW/1 -> est_quest_rp/3
  q_BN initial/1 -> q_BN_initial_unused/1

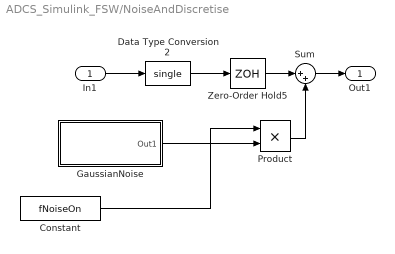
== system ADCS_Simulink_FSW/NoiseAndDiscretise ==
  In1 : Inport
  Constant : Constant  Value=fNoiseOn  OutDataTypeStr=single
  Data Type Conversion2 : DataTypeConversion  OutDataTypeStr=single  SaturateOnIntegerOverflow=off  RndMeth=Floor
  GaussianNoise : Subsystem  mask{Mean=Mean, Variance=Variance, dT=dT}
      mask prompts: dT "Sample Rate"
  Product : Product
  Sum : Sum  Inputs=|++
  Zero-Order Hold5 : ZeroOrderHold  SampleTime=dT
  Out1 : Outport
  wires:
  Data Type Conversion2/1 -> Zero-Order Hold5/1
  In1/1 -> Data Type Conversion2/1
  Sum/1 -> Out1/1
  Zero-Order Hold5/1 -> Sum/1
  GaussianNoise/1(Out1) -> Product/2
  Constant/1 -> Product/1
  Product/1 -> Sum/2

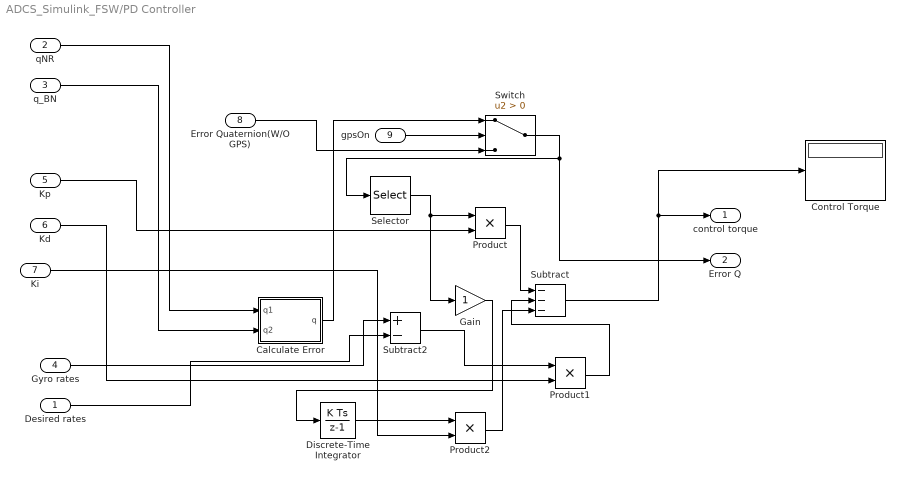
== system ADCS_Simulink_FSW/PD Controller ==
  Desired rates : Inport
  qNR : Inport  Port=2
  q_BN : Inport  Port=3
  Gyro rates : Inport  Port=4
  Kp : Inport  Port=5
  Kd : Inport  Port=6
  Ki : Inport  Port=7
  Error Quaternion(W/O GPS) : Inport  Port=8
  gpsOn : Inport  Port=9
  " Control Torque" : Display
  Calculate Error : MATLAB Function  TreatAsAtomicUnit=on
  Discrete-Time Integrator : DiscreteIntegrator  InitialCondition=[0;0;0]  SampleTime=0.1  ICPrevOutput=DiscIntNeverNeededParam  ICPrevScaledInput=DiscIntNeverNeededParam
  Gain : Gain
  Product : Product
  Product1 : Product
  Product2 : Product
  Selector : Selector  InputPortWidth=4  IndexOptions=Index vector (dialog)  Indices=[2 : 4]  OutputSizes=1
  Subtract : Sum  Inputs=---
  Subtract2 : Sum  Inputs=+-
  Switch : Switch  Criteria=u2 > Threshold  SaturateOnIntegerOverflow=off  InputSameDT=off
  control torque : Outport
  Error Q : Outport  Port=2
  wires:
  Selector/1 -> Gain/1, Product/1
  Product2/1 -> Subtract/3
  Product/1 -> Subtract/1
  Subtract2/1 -> Product1/1
  Discrete-Time Integrator/1 -> Product2/1
  Product1/1 -> Subtract/2
  Kp/1 -> Product/2
  Desired rates/1 -> Subtract2/2
  Kd/1 -> Product1/2
  Ki/1 -> Product2/2
  Gyro rates/1 -> Subtract2/1
  gpsOn/1 -> Switch/2
  Switch/1 -> Error Q/1, Selector/1
  Error Quaternion(W/O GPS)/1 -> Switch/3
  Gain/1 -> Discrete-Time Integrator/1
  Subtract/1 -> control torque/1, " Control Torque"/1
  q_BN/1 -> Calculate Error/2(q2)
  qNR/1 -> Calculate Error/1(q1)
  Calculate Error/1(q) -> Switch/1

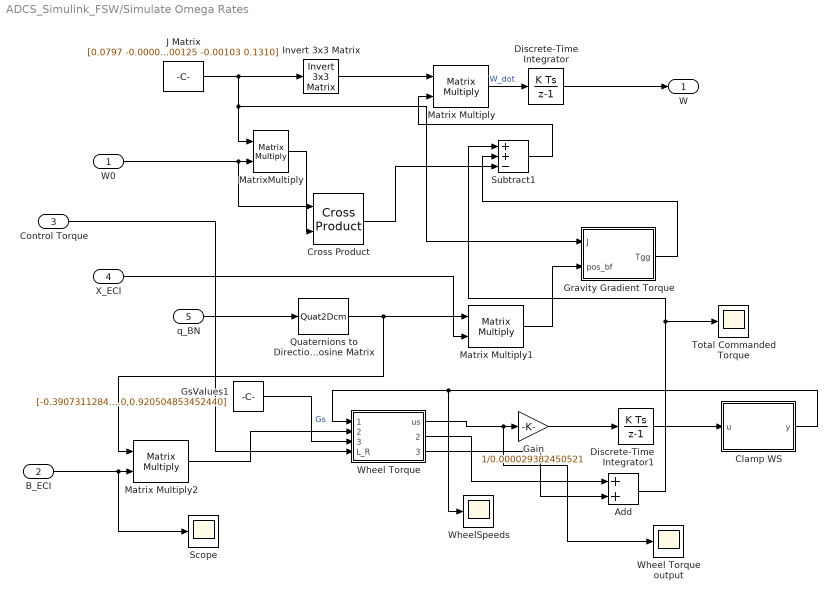
== system ADCS_Simulink_FSW/Simulate Omega Rates ==
  W0 : Inport
  "B_ECI " : Inport  Port=2
  Control Torque : Inport  Port=3
  X_ECI : Inport  Port=4
  q_BN : Inport  Port=5
  Add : Sum
  Clamp WS : MATLAB Function  TreatAsAtomicUnit=on
  Cross Product : matrix_library/Cross Product
  Discrete-Time Integrator : DiscreteIntegrator  gainval=1  InitialCondition=[0.12; -0.2; -0.05]  SampleTime=0.1  ICPrevOutput=DiscIntNeverNeededParam  ICPrevScaledInput=DiscIntNeverNeededParam
  Discrete-Time Integrator1 : DiscreteIntegrator  InitialCondition=[261.8; -261.8; 261.8; -261.8]  SampleTime=0.1  ICPrevOutput=DiscIntNeverNeededParam  ICPrevScaledInput=DiscIntNeverNeededParam
  Gain : Gain  Gain=1/0.000029382450521
  Gravity Gradient Torque : MATLAB Function  TreatAsAtomicUnit=on
  GsValues1 : Constant  Value=[-0.390731128489274,-0.390731128489274,0.390731128489274,0.390731128489274;0.0,0.920504853452440,0.920504853452440,0.0;0.920504853452440,0.0,0.0,0.920504853452440]
  Invert 3x3 Matrix : aerolibutil/Invert  3x3 Matrix
  J Matrix : Constant  Value=[0.0797 -0.00005 0.00125 ;-0.00005 0.1291 -0.00103;0.00125 -0.00103 0.1310]
  Matrix Multiply : Product  Multiplication=Matrix(*)
  Matrix Multiply1 : Product  Multiplication=Matrix(*)
  Matrix Multiply2 : Product  Multiplication=Matrix(*)
  MatrixMultiply : Product  Multiplication=Matrix(*)
  Quaternions to Direction Cosine Matrix : Quat2Dcm
  Scope : Scope
      settings: ActiveDisplayYMinimum=-20476.902247355712  ActiveDisplayYMaximum=14008.488779620786  DataLoggingVariableName=ScopeData27
  Subtract1 : Sum  Inputs=++-
  Total Commanded Torque : Scope
      settings: ActiveDisplayYMinimum=-0.0075192349082615706  ActiveDisplayYMaximum=0.0068794540520053359  DataLoggingVariableName=ScopeData7
  Wheel Torque : MATLAB Function  TreatAsAtomicUnit=on
  Wheel Torque output : Scope
      settings: ActiveDisplayYMinimum=-0.0066917259294539122  ActiveDisplayYMaximum=0.0049764737021494483  DataLoggingVariableName=ScopeData13
  WheelSpeeds : Scope
      settings: ActiveDisplayYMinimum=-114.37246424141858  ActiveDisplayYMaximum=1073.2158250334398  DataLoggingVariableName=ScopeData12
  W : Outport
  wires:
  Matrix Multiply/1 -> Discrete-Time Integrator/1  "W_dot"
  Cross Product/1 -> Subtract1/3
  Invert 3x3 Matrix/1 -> Matrix Multiply/1
  Control Torque/1 -> Wheel Torque/4(L_R)
  Subtract1/1 -> Matrix Multiply/2
  W0/1 -> Cross Product/1, MatrixMultiply/2
  Discrete-Time Integrator/1 -> W/1
  MatrixMultiply/1 -> Cross Product/2
  J Matrix/1 -> MatrixMultiply/1, Gravity Gradient Torque/1(J), Invert 3x3 Matrix/1
  X_ECI/1 -> Matrix Multiply1/2
  q_BN/1 -> Quaternions to Direction Cosine Matrix/1
  Quaternions to Direction Cosine Matrix/1 -> Matrix Multiply2/1, Matrix Multiply1/1
  Matrix Multiply1/1 -> Gravity Gradient Torque/2(pos_bf)
  GsValues1/1 -> Wheel Torque/3(GsValues)  "Gs"
  Wheel Torque/1(us) -> Wheel Torque output/1, Gain/1
  Gain/1 -> Discrete-Time Integrator1/1
  Discrete-Time Integrator1/1 -> Clamp WS/1(u)
  "B_ECI "/1 -> Scope/1, Matrix Multiply2/2
  Matrix Multiply2/1 -> Wheel Torque/2(mag_bf)
  Wheel Torque/2(tauMTB) -> Add/1
  Wheel Torque/3(t_3axis) -> Add/2
  Add/1 -> Subtract1/1, Total Commanded Torque/1
  Clamp WS/1(y) -> WheelSpeeds/1, Wheel Torque/1(wheel_speeds)
  Gravity Gradient Torque/1(Tgg) -> Subtract1/2

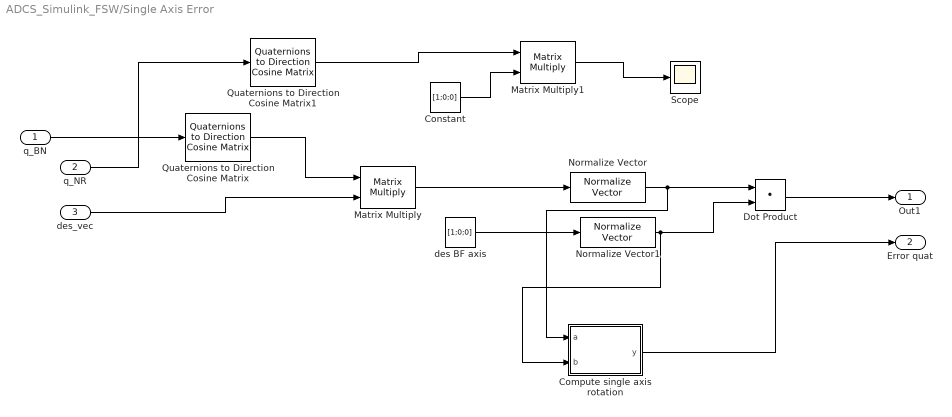
== system ADCS_Simulink_FSW/Single Axis Error ==
  q_BN : Inport
  q_NR : Inport  Port=2
  des_vec : Inport  Port=3
  Compute single axis rotation : MATLAB Function  TreatAsAtomicUnit=on
  Constant : Constant  Value=[1;0;0]
  Dot Product : DotProduct  OutDataTypeStr=Inherit: Inherit via internal rule
  Matrix Multiply : Product  Multiplication=Matrix(*)
  Matrix Multiply1 : Product  Multiplication=Matrix(*)
  Normalize Vector : vrlib/Utilities/Normalize Vector  maxzero=0
  Normalize Vector1 : vrlib/Utilities/Normalize Vector  maxzero=0
  Quaternions to Direction Cosine Matrix : sharedtransform/Quaternions to  Direction Cosine Matrix  aMode=aMode
      settings: LibrarySourceBlock=|
      | aerolibtransform2/Quaternions to
      | Direction Cosine Matrix
  Quaternions to Direction Cosine Matrix1 : sharedtransform/Quaternions to  Direction Cosine Matrix  aMode=aMode
      settings: LibrarySourceBlock=|
      | aerolibtransform2/Quaternions to
      | Direction Cosine Matrix
  Scope : Scope
      settings: ActiveDisplayYMinimum=-5.2569282896723637  ActiveDisplayYMaximum=4.2933395241699115  DataLoggingVariableName=ScopeData29
  des BF axis : Constant  Value=[1;0;0]
  Out1 : Outport
  Error quat : Outport  Port=2
  wires:
  q_BN/1 -> Quaternions to Direction Cosine Matrix/1
  des_vec/1 -> Matrix Multiply/2
  Normalize Vector1/1 -> Compute single axis rotation/2(b), Dot Product/2
  Normalize Vector/1 -> Compute single axis rotation/1(a), Dot Product/1
  Matrix Multiply/1 -> Normalize Vector/1
  des BF axis/1 -> Normalize Vector1/1
  Dot Product/1 -> Out1/1
  Compute single axis rotation/1(y) -> Error quat/1
  Quaternions to Direction Cosine Matrix/1 -> Matrix Multiply/1
  Constant/1 -> Matrix Multiply1/2
  Matrix Multiply1/1 -> Scope/1
  q_NR/1 -> Quaternions to Direction Cosine Matrix1/1
  Quaternions to Direction Cosine Matrix1/1 -> Matrix Multiply1/1

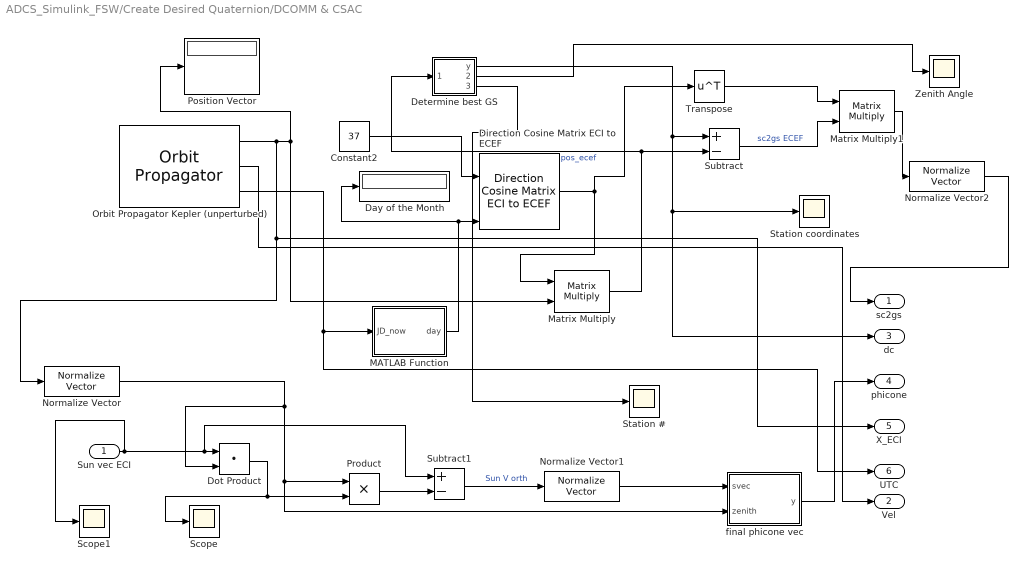
== system ADCS_Simulink_FSW/Create Desired Quaternion/DCOMM & CSAC ==
  Sun vec ECI : Inport
  Constant2 : Constant  Value=37
  Day of the Month : Display
  Determine best GS : MATLAB Function  TreatAsAtomicUnit=on
  Direction Cosine Matrix ECI to ECEF : aerolibtransform2/Direction Cosine Matrix ECI to ECEF  red=IAU-2000/2006  year=2025  month=October  day=7  hour=18  min=0  sec=0  deltaT=Day  errorflag=Error  extraparamflag=on
      settings: AttributesFormatString=%<red>
  Dot Product : DotProduct  OutDataTypeStr=Inherit: Inherit via internal rule
  MATLAB Function : MATLAB Function  TreatAsAtomicUnit=on
  Matrix Multiply : Product  Multiplication=Matrix(*)
  Matrix Multiply1 : Product  Multiplication=Matrix(*)
  Normalize Vector : vrlib/Utilities/Normalize Vector  maxzero=0
  Normalize Vector1 : vrlib/Utilities/Normalize Vector  maxzero=0
  Normalize Vector2 : vrlib/Utilities/Normalize Vector  maxzero=0
  Orbit Propagator Kepler (unperturbed) : OrbitPropagator  accelIn=on  startDate=juliandate(2025, 10, 7, 18, 0, 0)  semiMajorAxis=6821000  inclination=55  inertialPosition=[3649700.0 3308200.0 -4676600.0]  inertialVelocity=[-2750.8 6666.4 2573.4]  fixedPosition=[-4142689.0 -2676864.7 -4669861.6]  fixedVelocity=[1452.7 -6720.7 2568.1]  customR=3396200  customMu=4.305e13  customJ2=1.0826269e-03  customOmega=4.06125949e-3
  Position Vector : Display
  Product : Product
  Scope : Scope
      settings: ActiveDisplayYMinimum=-0.75552561150534214  ActiveDisplayYMaximum=-0.077868403904038916  DataLoggingVariableName=ScopeData9
  Scope1 : Scope
      settings: ActiveDisplayYMinimum=-1.8566059335886429  ActiveDisplayYMaximum=1.2542034832328808  DataLoggingVariableName=ScopeData10
  Station # : Scope
      settings: ActiveDisplayYMinimum=-3.9020645279013473  ActiveDisplayYMaximum=8.6314899749278684  DataLoggingVariableName=ScopeData17
  Station coordinates : Scope
      settings: ActiveDisplayYMinimum=-3.5092084454163194E+7  ActiveDisplayYMaximum=2.4351882117129691E+7  DataLoggingVariableName=ScopeData16
  Subtract : Sum  Inputs=+-
  Subtract1 : Sum  Inputs=+-
  Transpose : Math  Operator=transpose
  Zenith Angle : Scope
      settings: ActiveDisplayYMinimum=23.942233857370717  ActiveDisplayYMaximum=156.36741593298581  DataLoggingVariableName=ScopeData15
  final phicone vec : MATLAB Function  TreatAsAtomicUnit=on
  sc2gs : Outport
  Vel : Outport  Port=2
  dc : Outport  Port=3
  phicone : Outport  Port=4
  X_ECI : Outport  Port=5
  UTC : Outport  Port=6
  wires:
  Subtract/1 -> Matrix Multiply1/2  "sc2gs ECEF"
  Direction Cosine Matrix ECI to ECEF/1 -> Transpose/1, Matrix Multiply/1
  Determine best GS/1(y) -> dc/1, Station coordinates/1, Subtract/1
  Orbit Propagator Kepler (unperturbed)/1 -> Normalize Vector/1, X_ECI/1, Position Vector/1, Matrix Multiply/2
  Matrix Multiply/1 -> Subtract/2, Determine best GS/1(pos_ecef)  "pos_ecef"
  Constant2/1 -> Direction Cosine Matrix ECI to ECEF/2
  Sun vec ECI/1 -> Scope1/1, Subtract1/1, Dot Product/1
  Dot Product/1 -> Scope/1, Product/2
  Normalize Vector/1 -> Product/1, final phicone vec/2(zenith), Dot Product/2
  Product/1 -> Subtract1/2
  Subtract1/1 -> Normalize Vector1/1  "Sun V orth"
  Normalize Vector1/1 -> final phicone vec/1(svec)
  final phicone vec/1(y) -> phicone/1
  Transpose/1 -> Matrix Multiply1/1
  Matrix Multiply1/1 -> Normalize Vector2/1
  Normalize Vector2/1 -> sc2gs/1
  Orbit Propagator Kepler (unperturbed)/3 -> MATLAB Function/1(JD_now), UTC/1
  Determine best GS/2(bdangle) -> Zenith Angle/1
  Determine best GS/3(best) -> Station #/1
  MATLAB Function/1(day) -> Day of the Month/1, Direction Cosine Matrix ECI to ECEF/5
  Orbit Propagator Kepler (unperturbed)/2 -> Vel/1

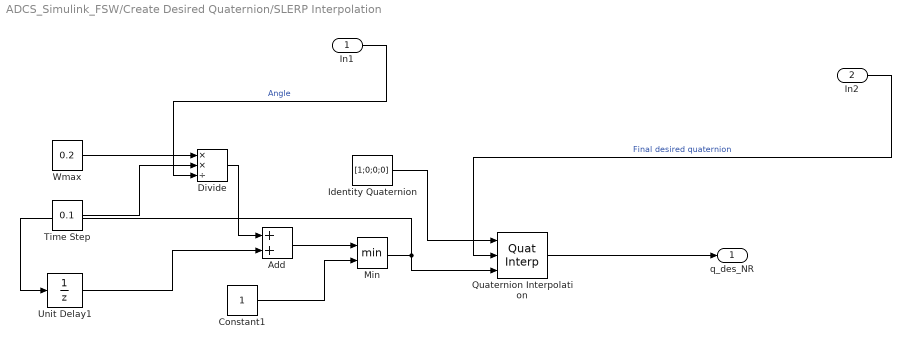
== system ADCS_Simulink_FSW/Create Desired Quaternion/SLERP Interpolation ==
  In1 : Inport
  In2 : Inport  Port=2
  Add : Sum
  Constant1 : Constant
  Divide : Product  Inputs=**/
  Identity Quaternion : Constant  Value=[1;0;0;0]
  Min : MinMax  Inputs=2
  Quaternion Interpolation : QuatInterp
  Time Step : Constant  Value=0.1
  Unit Delay1 : UnitDelay  SampleTime=-1  HasFrameUpgradeWarning=on
  Wmax : Constant  Value=0.2
  q_des_NR : Outport
  wires:
  Min/1 -> Quaternion Interpolation/3, Unit Delay1/1
  Unit Delay1/1 -> Add/2
  In2/1 -> Quaternion Interpolation/2  "Final desired quaternion"
  Identity Quaternion/1 -> Quaternion Interpolation/1
  Constant1/1 -> Min/2
  Time Step/1 -> Divide/2
  Wmax/1 -> Divide/1
  Divide/1 -> Add/1
  Add/1 -> Min/1
  Quaternion Interpolation/1 -> q_des_NR/1
  In1/1 -> Divide/3  "Angle"

== system ADCS_Simulink_FSW/Estimate Attitude/GaussianNoise ==
  Constant : Constant  Value=fUseNoise  VectorParams1D=off  OutDataTypeStr=single
  Data Type Conversion6 : DataTypeConversion  OutDataTypeStr=single  SaturateOnIntegerOverflow=off  RndMeth=Floor
  Product : Product
  Random Number : RandomNumber  Mean=Mean  Variance=Variance  Seed=randi([0 1000],size(Variance))  SampleTime=dT  VectorParams1D=off
  Out1 : Outport
  wires:
  Random Number/1 -> Data Type Conversion6/1
  Data Type Conversion6/1 -> Product/1
  Product/1 -> Out1/1
  Constant/1 -> Product/2
